simulink model "Lab3_p2_1_13b"  (R2013b)
settings: Solver=FixedStepDiscrete  SolverMode=SingleTasking  StartTime=0.0  StopTime=30  FixedStep=0.03  RelTol=1e-3
undefined symbols (not defined in the file): DiscIntNeverNeededParam
settings Model: SimulationMode=external  ExtModeTrigDuration=2  Creator=nding  LastModifiedBy=nding
settings OptimizationCC: OptimizeModelRefInitCode=on  LifeSpan=1
settings DebuggingCC: SolverPrmCheckMsg=none  InheritedTsInSrcMsg=none
settings HardwareCC: ProdBitPerInt=16  ProdBitPerPointer=8  ProdIntDivRoundTo=Zero  ProdEndianess=LittleEndian  ProdWordSize=8  ProdHWDeviceType=Atmel->AVR
settings RTWCC: SystemTargetFile=realtime.tlc  GenerateMakefile=off  TemplateMakefile=realtime.tmf  Description=Run on Target Hardware  RTWVerbose=off  ProcessScript=realtime_make_rtw_hook
settings STFCustomTargetCC: TargetLibSuffix=.a  GenerateSampleERTMain=on  ERTCustomFileBanners=on  SupportNonInlinedSFcns=off  SupportVariableSizeSignals=on  MATLABClassNameForMDSCustomization=Simulink.SoftwareTarget.ERTCustomization  GRTInterface=off  SystemTargetFile=realtime.tlc
settings ERTTargetCC: CodeReplacementLibrary=ANSI_C  GenerateSampleERTMain=on  ParMdlRefBuildCompliant=off  CompOptLevelCompliant=off  ConcurrentExecutionCompliant=off  CombineOutputUpdateFcns=off  ERTFirstTimeCompliant=off  SupportContinuousTime=on  SupportVariableSizeSignals=on  ModelStepFunctionPrototypeControlCompliant=off  CPPClassGenCompliant=off  ExtModeTransport=3  ExtModeMexFile=ext_serial_win32_comm  ExtModeMexArgs=0 1 9600  InlinedParameterPlacement=NonHierarchical  ERTSrcFileBannerTemplate=realtime_code_template.cgt  ERTHdrFileBannerTemplate=realtime_code_template.cgt  ERTDataSrcFileTemplate=realtime_code_template.cgt  ERTDataHdrFileTemplate=realtime_code_template.cgt  ERTCustomFileTemplate=realtime_file_process.tlc

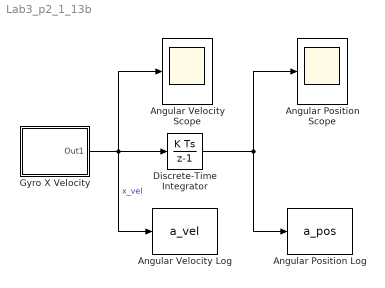
== system Lab3_p2_1_13b ==
  Angular Position Log : ToWorkspace  VariableName=a_pos  SampleTime=-1
  Angular Position Scope : Scope
      settings: YMin=-35000  YMax=35000
  Angular Velocity Log : ToWorkspace  VariableName=a_vel  SampleTime=-1
  Angular Velocity Scope : Scope
      settings: YMin=-35000  YMax=35000
  Discrete-Time Integrator : DiscreteIntegrator  SampleTime=-1  ICPrevOutput=DiscIntNeverNeededParam  ICPrevScaledInput=DiscIntNeverNeededParam
  Gyro X Velocity : Subsystem
  wires:
  Gyro X Velocity/1(Out1) -> Discrete-Time Integrator/1, Angular Velocity Log/1, Angular Velocity Scope/1  "x_vel"
  Discrete-Time Integrator/1 -> Angular Position Scope/1, Angular Position Log/1

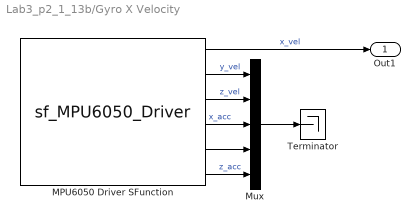
== system Lab3_p2_1_13b/Gyro X Velocity ==
  MPU6050 Driver SFunction : S-Function  InitFcn=try, set_param(gcb,'FunctionName','sf_MPU6050_Driver'), end  FunctionName=sf_MPU6050_Driver  SFunctionModules=sf_MPU6050_Driver_wrapper  EnableBusSupport=off  mask(S-Function Builder){}
      mask help: Simulink:masks:SFunctionBuilder_MD
      mask init:
      | val = [[.9  0.75 0.75 1 1 .9 .9 1]',[1 1 0.75 0.75 .9 .9 1 .9]'];try , sys = get_param(gcb,'SfunBuilderFcnName');if isempty(sys), sys = get_param(gcb,'FunctionName'); end,catch, sys = get_param(gcb,'FunctionName'); end
      settings: CopyFcn=set_param(gcbh,'LinkStatus','none')  PreSaveFcn=try, set_param(gcb,'FunctionName','sf_MPU6050_Driver'), end  OpenFcn=sfunctionwizard(gcbh)
      mask Display: plot(val(:,1),val(:,2)),disp(sys), port_label('output',1,'x_vel'), port_label('output',2,'y_vel'), port_label('output',3,'z_vel'), port_label('output',4,'x_acc'), port_label('output',5,'y_acc'), port_label('output',6,'z_acc')
  Mux : Mux  Inputs=5
  Terminator : Terminator
  Out1 : Outport
  wires:
  MPU6050 Driver SFunction/6 -> Mux/5  "z_acc"
  MPU6050 Driver SFunction/2 -> Mux/1  "y_vel"
  Mux/1 -> Terminator/1
  MPU6050 Driver SFunction/5 -> Mux/4
  MPU6050 Driver SFunction/3 -> Mux/2  "z_vel"
  MPU6050 Driver SFunction/4 -> Mux/3  "x_acc"
  MPU6050 Driver SFunction/1 -> Out1/1  "x_vel"
